simulink model "Central_Boost_MPPT_with_check"  (R2024b)
settings: Solver=FixedStepAuto  StartTime=0.0  StopTime=1  FixedStep=1e-6  RelTol=1e-3
libraries: spsSeriesRLCBranchLib x26, spsDiodeLib x13, spsPVArrayLib x12, spsVoltageMeasurementLib x3, spsControlledCurrentSourceLib x2, slpidlib x2, spsIGBTDiodeLib x1, spsCurrentMeasurementLib x1, spsPWMGeneratorDCDCLib x1, simulink x1, spspowerguiLib x1
settings Model: Creator=Nour Azzam  LastModifiedBy=Eng.Abd-Elrhman Saad

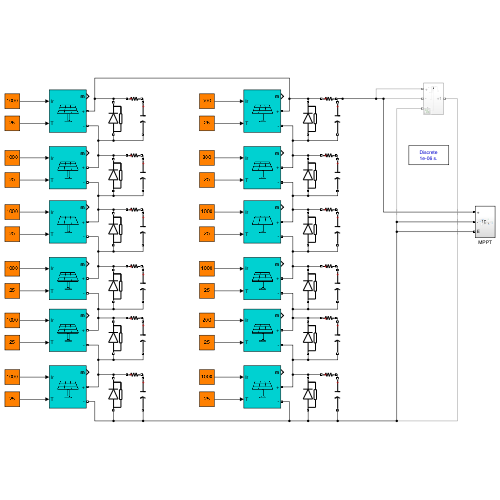
[thumbnail: Simulink's stored preview of the top-level diagram]
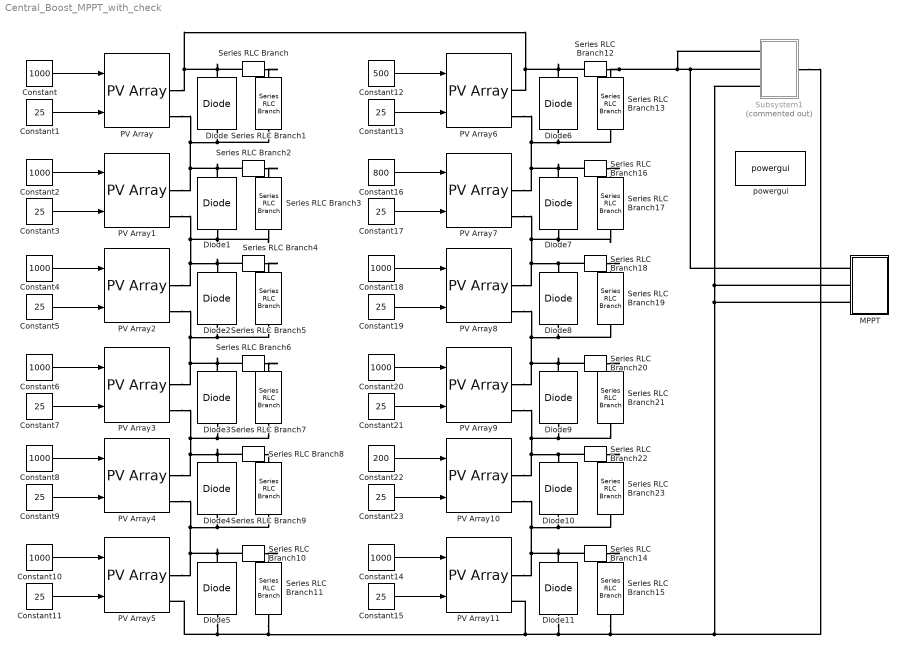
== system Central_Boost_MPPT_with_check ==
  Constant{,2,4,6,8,10,14,18,20} (9 alike) : Constant  Value=1000
  Constant{1,3,5,7,9,11,13,15,17,19,21,23} (12 alike) : Constant  Value=25
  Constant12 : Constant  Value=500
  Constant16 : Constant  Value=800
  Constant22 : Constant  Value=200
  Diode{,1..11} (12 alike) : spsDiodeLib/Diode  Ron=0.001  Lon=0  Vf=0.8  IC=0  UseSnubber=0  Rs=500  Cs=250e-9  Measurements=off
  MPPT : Subsystem
  PV Array{,1..11} (12 alike) : spsPVArrayLib/PV Array  Npar=1  Nser=1  PlotType=array @ 1000 W/m2 & specified temperatures  S_vec="[ 1000  500  100 ]"  Temp_C_vec="[ 45 25  ]"  ModuleName=User-defined  PlotWhenSelected=off  Pm=710.024  Ncell=60  Voc=49  Isc=18.4  Vm=40.9  Im=17.36  beta_Voc_pc=-0.36099  alpha_Isc_pc=0.102  beta_Voc=-0.17689  alpha_Isc=0.018768  IL=18.7149  I0=6.8806e-10  nI=1.3246  Rsh=89.315  Rs=0.11137  RobustModel=off  RobustCellTemperature=313.3991  BAL=on  Tc=1e-6  Tfilter=5e-5
  Series RLC Branch{,2,4,6,8,10,12,14,16,18,20,22} (12 alike) : spsSeriesRLCBranchLib/Series RLC Branch  LConnTagsString=__new0  RConnTagsString=__new0  BranchType=R  Resistance=0.01  Inductance=1e-3  SetiL0=off  InitialCurrent=0  Capacitance=1e-6  Setx0=off  InitialVoltage=0  Measurements=None
  Series RLC Branch{1,3,5,7,9,11,13,15,17,19,21,23} (12 alike) : spsSeriesRLCBranchLib/Series RLC Branch  LConnTagsString=__new0  RConnTagsString=__new0  BranchType=C  Resistance=1  Inductance=1e-3  SetiL0=off  InitialCurrent=0  Capacitance=10e-6  Setx0=off  InitialVoltage=0  Measurements=None
  Subsystem1 : Subsystem  Commented=on
  powergui : spspowerguiLib/powergui  Priority=1  SimulationMode=Discrete  SampleTime=1e-6  frequency=60  Iterations=50  frequencyindice=0  Pbase=100e6  ErrMax=1e-4  UnitsV=kV  UnitsW=MW  buscounter=0  FunctionMessages=off  echomessages=off  EnableUseOfTLC=off  CurrentSourceSwitches=off  DisableSnubberDevices=off  DisableRonSwitches=off  DisableVfSwitches=off  DisplayEquations=off  AutomaticDiscreteSolvers=off  SolverType=Tustin/Backward Euler (TBE)  Interpol=off  ExternalGateDelay=off  methode=off  Ts=100  x0status=blocks  SPID=on  SwTol=0  HookPort=off  NonlinearTolerance=1e-4  nMaxIteration=100  ContinueOnMaxIteration=off  RestoreLinks=warning  ResistiveCurrentMeasurement=off  Frange=[0:2:500]  Ylog=off  Xlog=on  ShowGrid=off  save=off  variable=ZData  structure=0  ZoomFFT=off  StartTime=0.0  cycles=1  DisplayStyle=1  fundamental=60  FreqAxis=off  MaxFrequency=1000  frequencyindicesteady=1  RmsSteady=1  display=off
  wires:
  Constant/1 -> PV Array/1
  Constant1/1 -> PV Array/2
  Constant2/1 -> PV Array1/1
  Constant3/1 -> PV Array1/2
  Constant7/1 -> PV Array3/2
  Constant6/1 -> PV Array3/1
  Constant4/1 -> PV Array2/1
  Constant5/1 -> PV Array2/2
  Constant11/1 -> PV Array5/2
  Constant10/1 -> PV Array5/1
  Constant8/1 -> PV Array4/1
  Constant9/1 -> PV Array4/2
  Constant12/1 -> PV Array6/1
  Constant16/1 -> PV Array7/1
  Constant19/1 -> PV Array8/2
  Constant18/1 -> PV Array8/1
  Constant21/1 -> PV Array9/2
  Constant14/1 -> PV Array11/1
  Constant15/1 -> PV Array11/2
  Constant17/1 -> PV Array7/2
  Constant23/1 -> PV Array10/2
  Constant20/1 -> PV Array9/1
  Constant22/1 -> PV Array10/1
  Constant13/1 -> PV Array6/2
  connections:
  Series RLC Branch/RConn1 -- Series RLC Branch1/LConn1
  PV Array1/RConn1 -- Diode1/RConn1 -- Series RLC Branch2/LConn1 -- PV Array/RConn2 -- Series RLC Branch1/RConn1 -- Diode/LConn1
  Series RLC Branch2/RConn1 -- Series RLC Branch3/LConn1
  Diode2/LConn1 -- Diode3/RConn1 -- Series RLC Branch6/LConn1 -- PV Array3/RConn1 -- PV Array2/RConn2 -- Series RLC Branch5/RConn1
  Diode2/RConn1 -- Diode1/LConn1 -- Series RLC Branch3/RConn1 -- PV Array1/RConn2 -- PV Array2/RConn1 -- Series RLC Branch4/LConn1
  Series RLC Branch6/RConn1 -- Series RLC Branch7/LConn1
  Series RLC Branch4/RConn1 -- Series RLC Branch5/LConn1
  Diode4/LConn1 -- Diode5/RConn1 -- Series RLC Branch10/LConn1 -- PV Array5/RConn1 -- PV Array4/RConn2 -- Series RLC Branch9/RConn1
  Diode4/RConn1 -- Diode3/LConn1 -- Series RLC Branch7/RConn1 -- PV Array3/RConn2 -- PV Array4/RConn1 -- Series RLC Branch8/LConn1
  Series RLC Branch10/RConn1 -- Series RLC Branch11/LConn1
  Series RLC Branch8/RConn1 -- Series RLC Branch9/LConn1
  Series RLC Branch14/LConn1 -- Diode10/LConn1 -- Series RLC Branch23/RConn1 -- PV Array10/RConn2 -- PV Array11/RConn1 -- Diode11/RConn1
  Series RLC Branch19/RConn1 -- Diode9/RConn1 -- Series RLC Branch20/LConn1 -- PV Array9/RConn1 -- PV Array8/RConn2 -- Diode8/LConn1
  PV Array10/RConn1 -- Diode9/LConn1 -- Series RLC Branch21/RConn1 -- PV Array9/RConn2 -- Series RLC Branch22/LConn1 -- Diode10/RConn1
  Series RLC Branch17/RConn1 -- Diode7/LConn1 -- PV Array7/RConn2 -- PV Array8/RConn1 -- Series RLC Branch18/LConn1 -- Diode8/RConn1
  Series RLC Branch16/LConn1 -- Diode7/RConn1 -- PV Array7/RConn1 -- PV Array6/RConn2 -- Series RLC Branch13/RConn1 -- Diode6/LConn1
  Series RLC Branch18/RConn1 -- Series RLC Branch19/LConn1
  Series RLC Branch12/RConn1 -- Subsystem1/LConn1 -- Subsystem1/LConn2 -- MPPT/LConn1 -- Series RLC Branch13/LConn1
  Series RLC Branch20/RConn1 -- Series RLC Branch21/LConn1
  Series RLC Branch22/RConn1 -- Series RLC Branch23/LConn1
  Series RLC Branch14/RConn1 -- Series RLC Branch15/LConn1
  Series RLC Branch16/RConn1 -- Series RLC Branch17/LConn1
  PV Array/RConn1 -- Diode/RConn1 -- Series RLC Branch/LConn1 -- Diode6/RConn1 -- Series RLC Branch12/LConn1 -- PV Array6/RConn1
  Diode5/LConn1 -- PV Array5/RConn2 -- Series RLC Branch11/RConn1 -- Subsystem1/RConn1 -- Subsystem1/LConn3 -- MPPT/LConn2 -- MPPT/LConn3 -- Series RLC Branch15/RConn1 -- Diode11/LConn1 -- PV Array11/RConn2

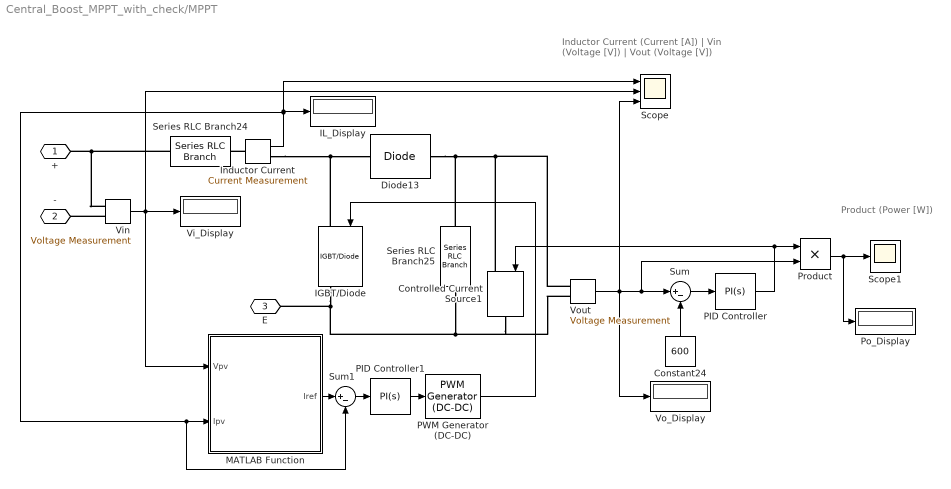
== system Central_Boost_MPPT_with_check/MPPT ==
  note: Inductor Current (Current [A]) |
      | Vin (Voltage [V]) | Vout (Voltage [V])
  note: Product (Power [W])
  Constant24 : Constant  Value=600
  Controlled Current Source1 : spsControlledCurrentSourceLib/Controlled Current Source  Initialize=off  Source_Type=AC  Amplitude=0  Phase=0  Frequency=0  Measurements=None
  Diode13 : spsDiodeLib/Diode  Ron=0.001  Lon=0  Vf=0.8  IC=0  UseSnubber=0  Rs=500  Cs=250e-9  Measurements=off
  IGBT/Diode : spsIGBTDiodeLib/IGBT//Diode  Ron=1e-3  Rs=1e5  Cs=inf  Measurements=on
  IL_Display : Display
  Inductor Current : spsCurrentMeasurementLib/Current Measurement  PhasorSimulation=off  OutputType=Complex  PSBequivalent=0
  MATLAB Function : MATLAB Function  TreatAsAtomicUnit=on
  PID Controller : slpidlib/PID Controller  Controller=PI  Form=Parallel  TimeDomain=Continuous-time  UseExternalTs=off  SampleTime=-1  IntegratorMethod=Forward Euler  FilterMethod=Forward Euler  ControllerParametersSource=internal  P=40.1047702980784  I=934.400726172757  UseKiTs=off  D=0  UseExternalDerivativeSource=off  N=100  UseFilter=on  TunerSelectOption=Transfer Function Based (PID Tuner App)  InitialConditionSource=internal  InitialConditionForIntegrator=0  InitialConditionForFilter=0  DifferentiatorICPrevScaledInput=0  ExternalReset=none  TrackingMode=off  Kt=1  LimitOutput=off  SatLimitsSource=internal  UpperSaturationLimit=0.95  LowerSaturationLimit=0  LinearizeAsGain=on  AntiWindupMode=clamping  Kb=1  LimitIntegrator=off  UpperIntegratorSaturationLimit=0.95  LowerIntegratorSaturationLimit=0  POutMin=[]  POutMax=[]  IOutMin=[]  IOutMax=[]  DOutMin=[]  DOutMax=[]  NOutMin=[]  NOutMax=[]  SumOutMin=[]  SumOutMax=[]  SaturationOutMin=[]  SaturationOutMax=[]  PParamMin=[]  PParamMax=[]  IParamMin=[]  IParamMax=[]  DParamMin=[]  DParamMax=[]  NParamMin=[]  NParamMax=[]  KbParamMin=[]  KbParamMax=[]  KtParamMin=[]  KtParamMax=[]  KbOutMin=[]  KbOutMax=[]  KtOutMin=[]  KtOutMax=[]  IntegratorOutMin=[]  IntegratorOutMax=[]  FilterOutMin=[]  FilterOutMax=[]  SumI1OutMin=[]  SumI1OutMax=[]  SumI2OutMin=[]  SumI2OutMax=[]  SumI3OutMin=[]  SumI3OutMax=[]  SumI4OutMin=[]  SumI4OutMax=[]  SumDOutMin=[]  SumDOutMax=[]  DifferentiatorOutMin=[]  DifferentiatorOutMax=[]  FilterDiffOutCoefMin=[]  FilterDiffOutCoefMax=[]  ReciprocalOutMin=[]  ReciprocalOutMax=[]  SumDenOutMin=[]  SumDenOutMax=[]  SumNumOutMin=[]  SumNumOutMax=[]  DivideOutMin=[]  DivideOutMax=[]  UdiffTsProdOutMin=[]  UdiffTsProdOutMax=[]  NTsProdOutMin=[]  NTsProdOutMax=[]  UintegralTsProdOutMin=[]  UintegralTsProdOutMax=[]  UngainTsProdOutMin=[]  UngainTsProdOutMax=[]  ClampingZeroOutDataTypeStr=Inherit: Inherit via back propagation  ClampingZeroOutMin=[]  ClampingZeroOutMax=[]  FilterDenConstantOutDataTypeStr=Inherit: Inherit via back propagation  FilterDenConstantOutMin=[]  FilterDenConstantOutMax=[]  PCopyOutDataTypeStr=Inherit: Inherit via back propagation  PCopyOutMin=[]  PCopyOutMax=[]  NCopyOutDataTypeStr=Inherit: Inherit via back propagation  NCopyOutMin=[]  NCopyOutMax=[]  IntegratorContinuousStateAttributes=''  IntegratorStateMustResolveToSignalObject=off  IntegratorRTWStateStorageClass=Auto  FilterContinuousStateAttributes=''  FilterStateMustResolveToSignalObject=off  FilterRTWStateStorageClass=Auto  ParallelPVariant=InternalParameters  IdealPVariant=Disabled  IVariant=InternalParameters  DVariant=Disabled  IntegratorVariant=Continuous  SatVariant=Disabled  AWVariant=Passthrough  PCopyVariant=Disabled  TRVariant=Disabled  FdbkBlocksVariant=Forward  IdealPFdbkVariant=Disabled  SatFdbkVariant=Disabled  DerivativeFilterVariant=Disabled  NVariant=Disabled  NCopyVariant=Disabled_SignalSpec  FilterICVariant=Disabled  IntegratorICVariant=InternalICs  ExternalResetVariant=Disabled  TRSumVariant=Passthrough  SumFdbkVariant=Disabled  SumVariant=Sum_PI  TsampFilterVariant=InternalTs  TsampNgainVariant=Passthrough  TsampIntegralVariant=Disabled_SignalSpec  ExternalSaturationOutDataTypeStr=Inherit: Same as second input  DerivativeSourceVariant=Disabled  PreIntVariant=InternalPreInt
  PID Controller1 : slpidlib/PID Controller  Controller=PI  Form=Parallel  TimeDomain=Continuous-time  UseExternalTs=off  SampleTime=-1  IntegratorMethod=Forward Euler  FilterMethod=Forward Euler  ControllerParametersSource=internal  P=0.05  I=10  UseKiTs=off  D=0  UseExternalDerivativeSource=off  N=100  UseFilter=on  TunerSelectOption=Transfer Function Based (PID Tuner App)  InitialConditionSource=internal  InitialConditionForIntegrator=0  InitialConditionForFilter=0  DifferentiatorICPrevScaledInput=0  ExternalReset=none  TrackingMode=off  Kt=1  LimitOutput=off  SatLimitsSource=internal  UpperSaturationLimit=0.85  LowerSaturationLimit=0.05  LinearizeAsGain=on  AntiWindupMode=clamping  Kb=1  LimitIntegrator=off  UpperIntegratorSaturationLimit=0.95  LowerIntegratorSaturationLimit=0  POutMin=[]  POutMax=[]  IOutMin=[]  IOutMax=[]  DOutMin=[]  DOutMax=[]  NOutMin=[]  NOutMax=[]  SumOutMin=[]  SumOutMax=[]  SaturationOutMin=[]  SaturationOutMax=[]  PParamMin=[]  PParamMax=[]  IParamMin=[]  IParamMax=[]  DParamMin=[]  DParamMax=[]  NParamMin=[]  NParamMax=[]  KbParamMin=[]  KbParamMax=[]  KtParamMin=[]  KtParamMax=[]  KbOutMin=[]  KbOutMax=[]  KtOutMin=[]  KtOutMax=[]  IntegratorOutMin=[]  IntegratorOutMax=[]  FilterOutMin=[]  FilterOutMax=[]  SumI1OutMin=[]  SumI1OutMax=[]  SumI2OutMin=[]  SumI2OutMax=[]  SumI3OutMin=[]  SumI3OutMax=[]  SumI4OutMin=[]  SumI4OutMax=[]  SumDOutMin=[]  SumDOutMax=[]  DifferentiatorOutMin=[]  DifferentiatorOutMax=[]  FilterDiffOutCoefMin=[]  FilterDiffOutCoefMax=[]  ReciprocalOutMin=[]  ReciprocalOutMax=[]  SumDenOutMin=[]  SumDenOutMax=[]  SumNumOutMin=[]  SumNumOutMax=[]  DivideOutMin=[]  DivideOutMax=[]  UdiffTsProdOutMin=[]  UdiffTsProdOutMax=[]  NTsProdOutMin=[]  NTsProdOutMax=[]  UintegralTsProdOutMin=[]  UintegralTsProdOutMax=[]  UngainTsProdOutMin=[]  UngainTsProdOutMax=[]  ClampingZeroOutDataTypeStr=Inherit: Inherit via back propagation  ClampingZeroOutMin=[]  ClampingZeroOutMax=[]  FilterDenConstantOutDataTypeStr=Inherit: Inherit via back propagation  FilterDenConstantOutMin=[]  FilterDenConstantOutMax=[]  PCopyOutDataTypeStr=Inherit: Inherit via back propagation  PCopyOutMin=[]  PCopyOutMax=[]  NCopyOutDataTypeStr=Inherit: Inherit via back propagation  NCopyOutMin=[]  NCopyOutMax=[]  IntegratorContinuousStateAttributes=''  IntegratorStateMustResolveToSignalObject=off  IntegratorRTWStateStorageClass=Auto  FilterContinuousStateAttributes=''  FilterStateMustResolveToSignalObject=off  FilterRTWStateStorageClass=Auto  ParallelPVariant=InternalParameters  IdealPVariant=Disabled  IVariant=InternalParameters  DVariant=Disabled  IntegratorVariant=Continuous  SatVariant=Disabled  AWVariant=Passthrough  PCopyVariant=Disabled  TRVariant=Disabled  FdbkBlocksVariant=Forward  IdealPFdbkVariant=Disabled  SatFdbkVariant=Disabled  DerivativeFilterVariant=Disabled  NVariant=Disabled  NCopyVariant=Disabled_SignalSpec  FilterICVariant=Disabled  IntegratorICVariant=InternalICs  ExternalResetVariant=Disabled  TRSumVariant=Passthrough  SumFdbkVariant=Disabled  SumVariant=Sum_PI  TsampFilterVariant=InternalTs  TsampNgainVariant=Passthrough  TsampIntegralVariant=Disabled_SignalSpec  ExternalSaturationOutDataTypeStr=Inherit: Same as second input  DerivativeSourceVariant=Disabled  PreIntVariant=InternalPreInt
  PWM Generator (DC-DC) : spsPWMGeneratorDCDCLib/PWM Generator (DC-DC)  Fsw=10000  Ts=0
  Po_Display : Display
  Product : Product
  Scope : Scope  NumInputPorts=3
  Scope1 : Scope
  Series RLC Branch24 : spsSeriesRLCBranchLib/Series RLC Branch  LConnTagsString=__new0  RConnTagsString=__new0  BranchType=L  Resistance=1  Inductance=20e-3  SetiL0=off  InitialCurrent=0  Capacitance=10e-6  Setx0=off  InitialVoltage=0  Measurements=None
  Series RLC Branch25 : spsSeriesRLCBranchLib/Series RLC Branch  LConnTagsString=__new0  RConnTagsString=__new0  BranchType=C  Resistance=1  Inductance=5e-3  SetiL0=off  InitialCurrent=0  Capacitance=30e-3  Setx0=on  InitialVoltage=600  Measurements=None
  Sum : Sum  Inputs=|+-
  Sum1 : Sum  Inputs=|+-
  Vi_Display : Display
  Vin : spsVoltageMeasurementLib/Voltage Measurement  PhasorSimulation=off  OutputType=Complex  PSBequivalent=0
  Vo_Display : Display
  Vout : spsVoltageMeasurementLib/Voltage Measurement  PhasorSimulation=off  OutputType=Complex  PSBequivalent=0
  + : PMIOPort  Side=Left
  - : PMIOPort  Port=2  Side=Left
  E : PMIOPort  Port=3  Side=Left
  wires:
  Sum/1 -> PID Controller/1
  Sum1/1 -> PID Controller1/1
  PID Controller/1 -> Controlled Current Source1/1, Product/1
  MATLAB Function/1(Iref) -> Sum1/1
  PID Controller1/1 -> PWM Generator (DC-DC)/1
  Vin/1 -> MATLAB Function/1(Vpv), Vi_Display/1, Scope/2
  Product/1 -> Po_Display/1, Scope1/1
  Inductor Current/1 -> Scope/1, IL_Display/1, Sum1/2, MATLAB Function/2(Ipv)
  PWM Generator (DC-DC)/1 -> IGBT/Diode/1
  Vout/1 -> Vo_Display/1, Product/2, Sum/1, Scope/3
  Constant24/1 -> Sum/2
  connections:
  Series RLC Branch24/RConn1 -- +/RConn1 -- Vin/LConn1
  Diode13/RConn1 -- Series RLC Branch25/LConn1 -- Vout/LConn1 -- Controlled Current Source1/LConn1
  Inductor Current/LConn1 -- Series RLC Branch24/LConn1
  Inductor Current/RConn1 -- IGBT/Diode/LConn1 -- Diode13/LConn1
  Series RLC Branch25/RConn1 -- Vout/LConn2 -- Controlled Current Source1/RConn1 -- IGBT/Diode/RConn1 -- E/RConn1
  Vin/LConn2 -- -/RConn1

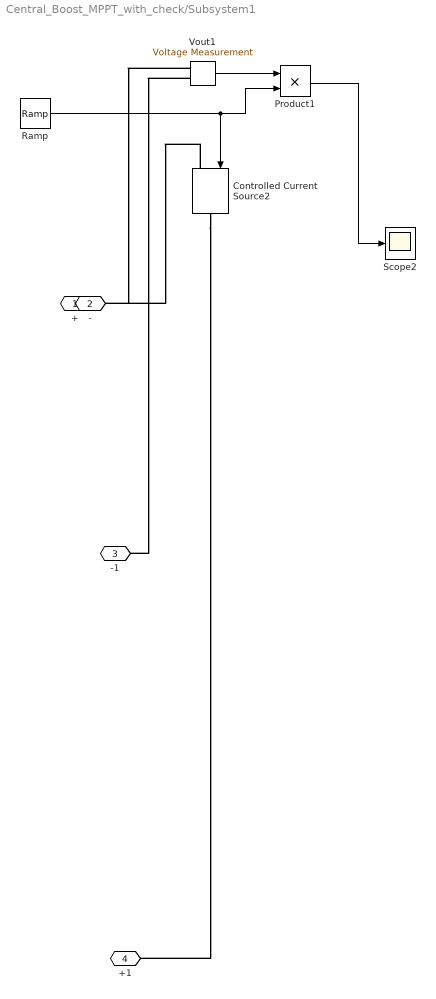
== system Central_Boost_MPPT_with_check/Subsystem1 ==
  Controlled Current Source2 : spsControlledCurrentSourceLib/Controlled Current Source  Initialize=off  Source_Type=AC  Amplitude=0  Phase=0  Frequency=0  Measurements=None
  Product1 : Product
  Ramp : simulink/Sources/Ramp  slope=18.4*2  start=0  InitialOutput=0
  Scope2 : Scope
  Vout1 : spsVoltageMeasurementLib/Voltage Measurement  PhasorSimulation=off  OutputType=Complex  PSBequivalent=0
  + : PMIOPort  Side=Left
  - : PMIOPort  Port=2  Side=Left
  -1 : PMIOPort  Port=3  Side=Left
  +1 : PMIOPort  Port=4  Side=Right
  wires:
  Product1/1 -> Scope2/1
  Vout1/1 -> Product1/1
  Ramp/1 -> Product1/2, Controlled Current Source2/1
  connections:
  Vout1/LConn1 -- +/RConn1
  Vout1/LConn2 -- -1/RConn1
  Controlled Current Source2/RConn1 -- +1/RConn1
  Controlled Current Source2/LConn1 -- -/RConn1

== matlab function Central_Boost_MPPT_with_check/MPPT/MATLAB Function ==
  settings: updateMethod=DISCRETE
  data: Vpv input; Iref output; Ipv input
function Iref = mppt_global_forced(Vpv, Ipv)
    persistent V_target Pmax Vbest mode timer;
    
    Ts = 1e-6;
    
    % Voltage sweep parameters - sweep Vpv from high to low
    V_oc_est = 300;           % Estimated open circuit voltage
    V_scan_min = 240;         % Minimum scan voltage
    V_ramp_rate = 150;        % V/s sweep rate
    
    if isempty(V_target)
        V_target = V_oc_est;
        Pmax = 0;
        Vbest = 240;          % Start with nominal MPP voltage
        mode = 0;
        timer = 0;
    end
    
    Ppv = Vpv * Ipv;
    
    switch mode
        case 0  % RESET - go to high voltage (low current)
            V_target = V_oc_est;
            Pmax = 0;
            if Vpv > 245       % Near Voc
                mode = 1;
            end
            
        case 1  % SCAN - sweep voltage DOWN to find global Pmax
            % Record power at each voltage
            if Ppv > Pmax
                Pmax = Ppv;
                Vbest = V_target;
            end
            
            V_target = V_target - (V_ramp_rate * Ts);
            
            if V_target <= V_scan_min
                mode = 2;
            end
            
        case 2  % RETURN to Vbest
            if V_target < Vbest
                V_target = V_target + (300 * Ts);
            else
                V_target = Vbest;
                mode = 3;
                timer = 0;
            end
            
        case 3  % HOLD
            timer = timer + Ts;
            if timer >= 1.0
                mode = 0;
            end
    end
    
    % INNER LOOP: Current controller to regulate Vpv to V_target
    % Simple P-control: if Vpv > V_target, increase current (load more)
    %                  if Vpv < V_target, decrease current (load less)
    persistent err_int;
    if isempty(err_int), err_int = 0; end
    
    err = Vpv - V_target;           % Positive = need more load
    err_int = err_int + err * Ts;
    err_int = max(min(err_int, 50), -50);  % Anti-windup
    
    Kp = 1;   % Proportional gain
    Ki = 200;   % Integral gain
    
    % Base current + correction
    I_calc = 20 + Kp * err + Ki * err_int;
    
    % Limit output
    Iref = max(min(I_calc, 35), 0);
end
